simulink model "TestModel_V5_Timing_2024a"  (R2024a)
settings: Solver=FixedStepAuto  StartTime=0.0  StopTime=40  FixedStep=1e-6  RelTol=1e-3
values from neighbouring files (symbols this model uses):
  par_Ctrl_FluxOffset = 0    [Param.m]
  par_Ctrl_MI = 0.99    [Param.m]
  par_Ctrl_SpdRt = 10    [Param.m]
  par_Ctrl_ThetaOffset = 0    [Param.m]
  par_IM_Frated = 50    [Param.m]
  par_IM_IratedPh = 7.9/sqrt(3)    [Param.m]
  par_IM_Lm = 0.527    [Param.m]
  par_IM_Lr = par_IM_Lm + par_IM_Llr    (= 0.5639)    [Param.m]
  par_IM_pp = 2    [Param.m]
  par_IM_Rs = 3.14    [Param.m]
  par_IM_VrmsLL = 400    [Param.m]
  par_uc_Ts = 100e-6    (= 0.0001)    [Param.m]
  pmsm = mcb.getPMSMParameters('Teknic2310P')    [mcb_pmsm_foc_sensorless_f28379d_datascript.m]
  Ts = T_pwm    (= 5e-05)    [mcb_pmsm_foc_sensorless_f28379d_datascript.m]
  Ts_motor = T_pwm/2    (= 2.5e-05)    [mcb_pmsm_foc_sensorless_f28379d_datascript.m]
undefined symbols (not defined in the file or in its folder): DiscIntNeverNeededParam, IM, par_pmsm_FluxLinkage, par_pmsm_Frated, par_pmsm_pp, par_pmsm_Vboost, par_pmsm_VrmsLL
libraries: spsOnDelayLib x24, mcbcontrolslib x11, spsTriangleGeneratorLib x4, autolibim x3, spsCurrentMeasurementLib x2, spsDCVoltageSourceLib x2, spsVoltageMeasurementLib x2, spsTwoLevelConverterLib x2, spsThreePhaseVIMeasurementLib x2, spsSeriesRLCBranchLib x1, sdolib x1, spsUniversalBridgeLib x1
(part 2 of 3)

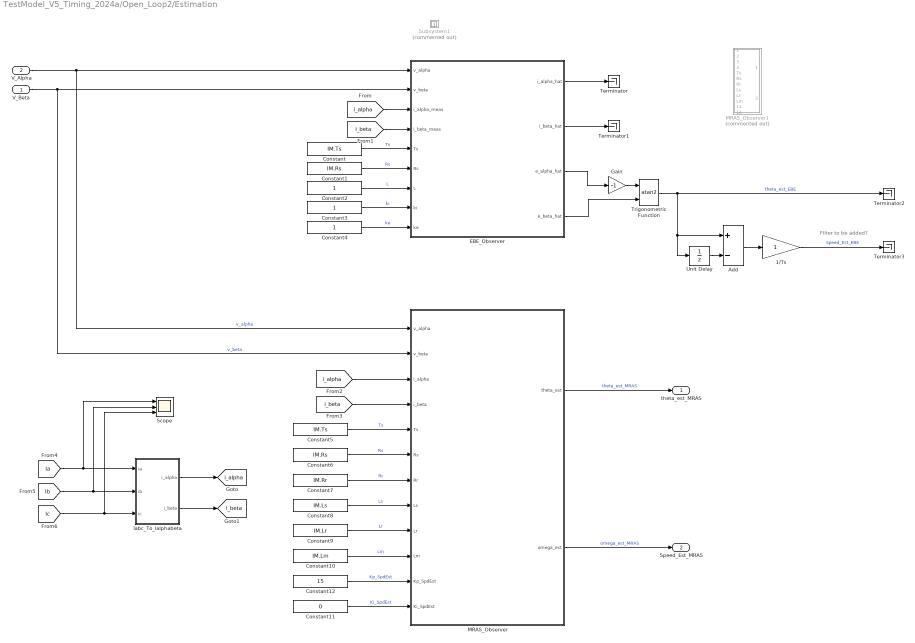
== system TestModel_V5_Timing_2024a/Open_Loop2/Estimation ==
  note: Filter to be added?
  V_Beta : Inport
  V_Alpha : Inport  Port=2
  1/Ts : Gain
  Add : Sum  Inputs=+-
  Constant : Constant  Value=IM.Ts
  Constant1 : Constant  Value=IM.Rs
  Constant10 : Constant  Value=IM.Lm
  Constant11 : Constant  Value=0
  Constant12 : Constant  Value=15
  Constant2 : Constant
  Constant3 : Constant
  Constant4 : Constant
  Constant5 : Constant  Value=IM.Ts
  Constant6 : Constant  Value=IM.Rs
  Constant7 : Constant  Value=IM.Rr
  Constant8 : Constant  Value=IM.Ls
  Constant9 : Constant  Value=IM.Lr
  EBE_Observer : MATLAB Function  TreatAsAtomicUnit=on
  Gain : Gain  Gain=-1
  Iabc_To_Ialphabeta : Subsystem
  MRAS_Observer : MATLAB Function  TreatAsAtomicUnit=on
  MRAS_Observer1 : MATLAB Function  Commented=on  TreatAsAtomicUnit=on
  Scope : Scope  NumInputPorts=3
  Subsystem1 : Subsystem  Commented=on
  Terminator{,1..3} (4 alike) : Terminator
  Trigonometric Function : Trigonometry  Operator=atan2
  Unit Delay : UnitDelay  SampleTime=-1  HasFrameUpgradeWarning=on
  theta_est_MRAS : Outport  VectorParamsAs1DForOutWhenUnconnected=off
  Speed_Est_MRAS : Outport  Port=2  VectorParamsAs1DForOutWhenUnconnected=off
  tag scope: i_alpha=global, i_beta=global
  wires:
  [Ia] -> Scope/1, Iabc_To_Ialphabeta/1(ia)
  [Ib] -> Scope/2, Iabc_To_Ialphabeta/2(ib)
  [Ic] -> Scope/3, Iabc_To_Ialphabeta/3(ic)
  Iabc_To_Ialphabeta/1(i_alpha) -> [i_alpha]
  Iabc_To_Ialphabeta/2(i_beta) -> [i_beta]
  V_Alpha/1 -> MRAS_Observer/1(v_alpha), EBE_Observer/1(v_alpha)  "v_alpha"
  V_Beta/1 -> MRAS_Observer/2(v_beta), EBE_Observer/2(v_beta)  "v_beta"
  Constant/1 -> EBE_Observer/5(Ts)  "Ts"
  Constant1/1 -> EBE_Observer/6(Rs)  "Rs"
  Constant2/1 -> EBE_Observer/7(L)  "L"
  Constant3/1 -> EBE_Observer/8(ki)  "ki"
  Constant4/1 -> EBE_Observer/9(ke)  "ke"
  EBE_Observer/3(e_alpha_hat) -> Gain/1
  Gain/1 -> Trigonometric Function/1
  EBE_Observer/4(e_beta_hat) -> Trigonometric Function/2
  Trigonometric Function/1 -> Terminator2/1, Unit Delay/1, Add/1  "theta_est_EBE"
  Unit Delay/1 -> Add/2
  Add/1 -> 1/Ts/1
  1/Ts/1 -> Terminator3/1  "Speed_Est_EBE"
  EBE_Observer/1(i_alpha_hat) -> Terminator/1
  EBE_Observer/2(i_beta_hat) -> Terminator1/1
  [i_alpha] -> EBE_Observer/3(i_alpha_meas)
  [i_beta] -> EBE_Observer/4(i_beta_meas)
  [i_alpha] -> MRAS_Observer/3(i_alpha)
  [i_beta] -> MRAS_Observer/4(i_beta)
  Constant9/1 -> MRAS_Observer/9(Lr)  "Lr"
  Constant7/1 -> MRAS_Observer/7(Rr)  "Rr"
  Constant6/1 -> MRAS_Observer/6(Rs)  "Rs"
  Constant5/1 -> MRAS_Observer/5(Ts)  "Ts"
  Constant10/1 -> MRAS_Observer/10(Lm)  "Lm"
  Constant12/1 -> MRAS_Observer/11(Kp_SpdEst)  "Kp_SpdEst"
  Constant11/1 -> MRAS_Observer/12(Ki_SpdEst)  "Ki_SpdEst"
  MRAS_Observer/1(theta_est) -> theta_est_MRAS/1  "theta_est_MRAS"
  MRAS_Observer/2(omega_est) -> Speed_Est_MRAS/1  "omega_est_MRAS"
  Constant8/1 -> MRAS_Observer/8(Ls)  "Ls"

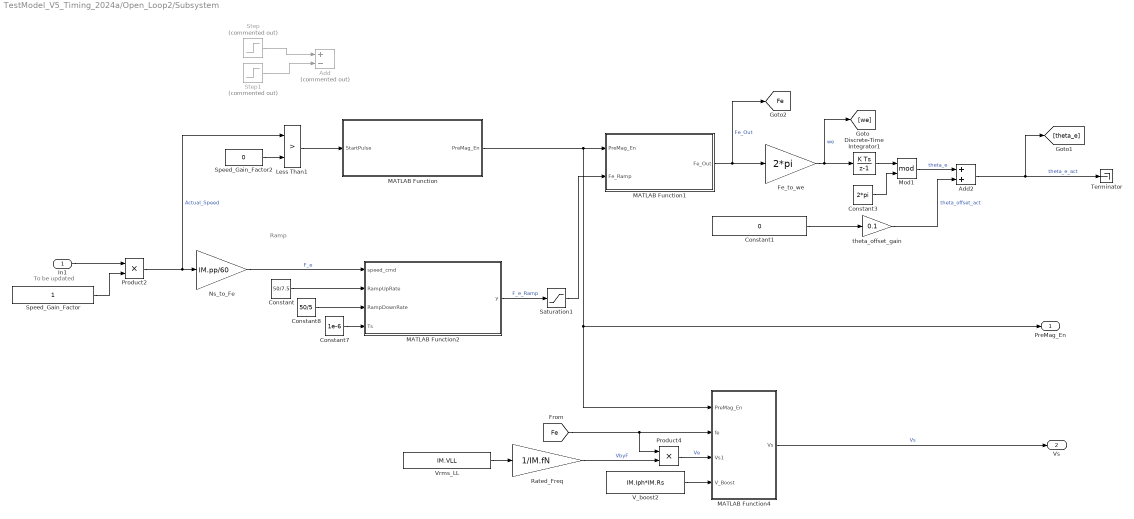
== system TestModel_V5_Timing_2024a/Open_Loop2/Subsystem ==
  note: To be updated
  note: Ramp
  In1 : Inport
  Add : Sum  Commented=on  Inputs=+-
  Add2 : Sum
  Constant : Constant  Value=50/7.5
  Constant1 : Constant  Value=0
  Constant3 : Constant  Value=2*pi  OutDataTypeStr=double
  Constant7 : Constant  Value=1e-6
  Constant8 : Constant  Value=50/5
  Discrete-Time Integrator1 : DiscreteIntegrator  SampleTime=-1  OutDataTypeStr=double  ICPrevOutput=DiscIntNeverNeededParam  ICPrevScaledInput=DiscIntNeverNeededParam
  Fe_to_we : Gain  Gain=2*pi
  Less Than1 : RelationalOperator  Operator=>  OutDataTypeStr=boolean  RndMeth=Simplest  InputSameDT=off
  MATLAB Function : MATLAB Function  TreatAsAtomicUnit=on
  MATLAB Function1 : MATLAB Function  TreatAsAtomicUnit=on
  MATLAB Function2 : MATLAB Function  TreatAsAtomicUnit=on
  MATLAB Function4 : MATLAB Function  TreatAsAtomicUnit=on
  Mod1 : Math  Operator=mod
  Ns_to_Fe : Gain  Gain=IM.pp/60
  Product2 : Product
  Product4 : Product
  Rated_Freq : Gain  Gain=1/IM.fN  ParamDataTypeStr=double  OutDataTypeStr=double
  Saturation1 : Saturate  UpperLimit=50  LowerLimit=0
  Speed_Gain_Factor : Constant
  Speed_Gain_Factor2 : Constant  Value=0
  Step : Step  Commented=on
  Step1 : Step  Commented=on  Time=1.2
  Terminator : Terminator
  V_boost2 : Constant  Value=IM.Iph*IM.Rs
  Vrms_LL : Constant  Value=IM.VLL  OutDataTypeStr=double
  theta_offset_gain : Gain  Gain=0.1
  PreMag_En : Outport  VectorParamsAs1DForOutWhenUnconnected=off
  Vs : Outport  Port=2  VectorParamsAs1DForOutWhenUnconnected=off
  tag scope: Fe=global
  wires:
  Step1/1 -> Add/2
  Add2/1 -> Terminator/1, [theta_e]  "theta_e_act"
  Discrete-Time Integrator1/1 -> Mod1/1
  Product2/1 -> Ns_to_Fe/1, Less Than1/1  "Actual_Speed"
  MATLAB Function/1(PreMag_En) -> MATLAB Function4/1(PreMag_En), PreMag_En/1, MATLAB Function1/1(PreMag_En)
  [Fe] -> MATLAB Function4/2(fe), Product4/1
  Product4/1 -> MATLAB Function4/3(Vs1)  "Ve"
  Constant1/1 -> theta_offset_gain/1
  Rated_Freq/1 -> Product4/2  "VbyF"
  V_boost2/1 -> MATLAB Function4/4(V_Boost)
  MATLAB Function1/1(Fe_Out) -> [Fe], Fe_to_we/1  "Fe_Out"
  Constant/1 -> MATLAB Function2/2(RampUpRate)
  Fe_to_we/1 -> Discrete-Time Integrator1/1, [we]  "we"
  Constant7/1 -> MATLAB Function2/4(Ts)
  Less Than1/1 -> MATLAB Function/1(StartPulse)
  Saturation1/1 -> MATLAB Function1/2(Fe_Ramp)
  Ns_to_Fe/1 -> MATLAB Function2/1(speed_cmd)  "F_e"
  Step/1 -> Add/1
  Speed_Gain_Factor2/1 -> Less Than1/2
  Speed_Gain_Factor/1 -> Product2/2
  Constant8/1 -> MATLAB Function2/3(RampDownRate)
  MATLAB Function4/1(Vs) -> Vs/1  "Vs"
  Mod1/1 -> Add2/1  "theta_e"
  MATLAB Function2/1(y) -> Saturation1/1  "F_e_Ramp"
  Constant3/1 -> Mod1/2
  theta_offset_gain/1 -> Add2/2  "theta_offset_act"
  Vrms_LL/1 -> Rated_Freq/1
  In1/1 -> Product2/1

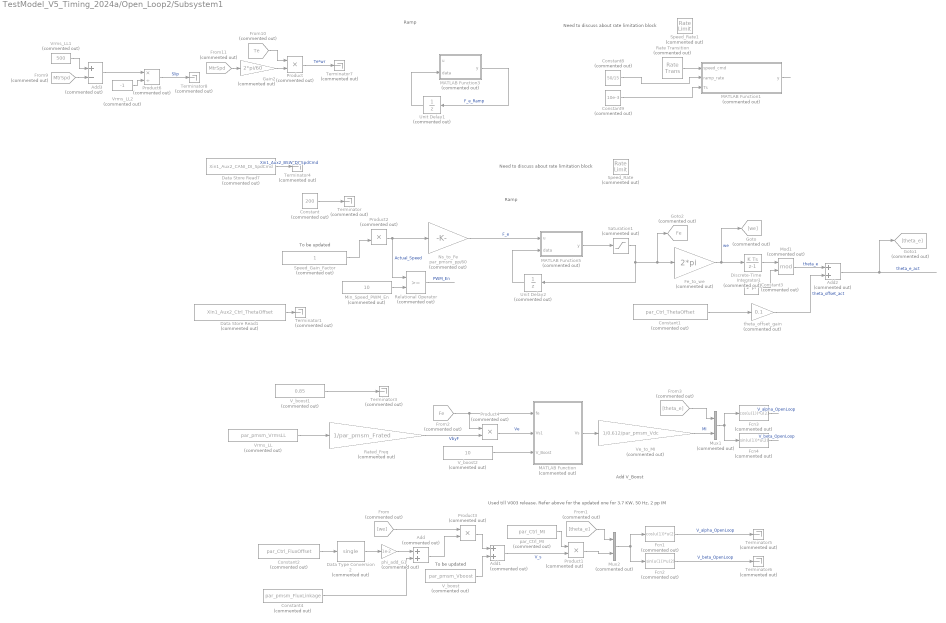
== system TestModel_V5_Timing_2024a/Open_Loop2/Subsystem1 ==
  note: Add V_Boost
  note: Used till V003 release. Refer above for the updated one for 3.7 KW, 50 Hz, 2 pp IM
  note: Ramp
  note: Need to discuss about rate limitation block
  note: To be updated
  note: To be updated
  note: Need to discuss about rate limitation block
  note: Ramp
  Add : Sum  Commented=on
  Add1 : Sum  Commented=on
  Add2 : Sum  Commented=on
  Add3 : Sum  Commented=on  Inputs=+-
  Constant : Constant  Commented=on  Value=200
  Constant1 : Constant  Commented=on  Value=par_Ctrl_ThetaOffset
  Constant2 : Constant  Commented=on  Value=par_Ctrl_FluxOffset
  Constant3 : Constant  Commented=on  Value=2*pi  OutDataTypeStr=double
  Constant4 : Constant  Commented=on  Value=par_pmsm_FluxLinkage  OutDataTypeStr=double
  Constant8 : Constant  Commented=on  Value=50/15
  Constant9 : Constant  Commented=on  Value=10e-3
  Data Store Read1 : DataStoreRead  Commented=on  DataStoreName=Xin1_Aux2_Ctrl_ThetaOffset  IndexOptions=Index vector (dialog)  Indices=1  OutputSizes=1
  Data Store Read7 : DataStoreRead  Commented=on  DataStoreName=Xin1_Aux2_CANI_DI_SpdCmd  IndexOptions=Index vector (dialog)  Indices=1  OutputSizes=1
  Data Type Conversion2 : DataTypeConversion  Commented=on  OutDataTypeStr=single  SaturateOnIntegerOverflow=off  RndMeth=Floor
  Discrete-Time Integrator1 : DiscreteIntegrator  Commented=on  SampleTime=-1  OutDataTypeStr=double  ICPrevOutput=DiscIntNeverNeededParam  ICPrevScaledInput=DiscIntNeverNeededParam
  Fcn1 : Fcn  Commented=on  Expr=cos(u(1))*u(2)
  Fcn2 : Fcn  Commented=on  Expr=sin(u(1))*u(2)
  Fcn3 : Fcn  Commented=on  Expr=cos(u(1))*u(2)
  Fcn4 : Fcn  Commented=on  Expr=sin(u(1))*u(2)
  Fe_to_we : Gain  Commented=on  Gain=2*pi
  From : From  Commented=on  GotoTag=we
  From1 : From  Commented=on  GotoTag=theta_e
  From10 : From  Commented=on  GotoTag=Te
  From11 : From  Commented=on  GotoTag=MtrSpd
  From2 : From  Commented=on  GotoTag=Fe  TagVisibility=global
  From3 : From  Commented=on  GotoTag=theta_e
  From9 : From  Commented=on  GotoTag=MtrSpd
  Gain2 : Gain  Commented=on  Gain=2*pi/60
  Goto : Goto  Commented=on  GotoTag=we
  Goto1 : Goto  Commented=on  GotoTag=theta_e
  Goto2 : Goto  Commented=on  GotoTag=Fe  TagVisibility=global
  MATLAB Function : MATLAB Function  Commented=on  TreatAsAtomicUnit=on
  MATLAB Function1 : MATLAB Function  Commented=on  TreatAsAtomicUnit=on
  MATLAB Function3 : MATLAB Function  Commented=on  TreatAsAtomicUnit=on
  MATLAB Function5 : MATLAB Function  Commented=on  TreatAsAtomicUnit=on
  Min_Speed_PWM_En : Constant  Commented=on  Value=10
  Mod1 : Math  Commented=on  Operator=mod
  Mux1 : Mux  Commented=on  Inputs=2
  Mux2 : Mux  Commented=on  Inputs=2
  Ns_to_Fe : Gain  Commented=on  Gain=par_pmsm_pp/60
  Product{,1..4} (5 alike) : Product  Commented=on
  Product6 : Product  Commented=on  Inputs=*/
  Rate Transition : RateTransition  Commented=on  OutPortSampleTime=10e-3
  Rated_Freq : Gain  Commented=on  Gain=1/par_pmsm_Frated  ParamDataTypeStr=double  OutDataTypeStr=double
  Relational Operator : RelationalOperator  Commented=on  OutDataTypeStr=boolean  RndMeth=Simplest  InputSameDT=off
  Saturation1 : Saturate  Commented=on  UpperLimit=50  LowerLimit=0
  Speed_Gain_Factor : Constant  Commented=on
  Speed_Rate : RateLimiter  Commented=on  RisingSlewLimit=par_Ctrl_SpdRt  FallingSlewLimit=-par_Ctrl_SpdRt  SampleTimeMode=inherited
  Speed_Rate1 : RateLimiter  Commented=on  RisingSlewLimit=par_Ctrl_SpdRt  FallingSlewLimit=-par_Ctrl_SpdRt  SampleTimeMode=inherited
  Terminator{,1,3..8} (8 alike) : Terminator  Commented=on
  Unit Delay1 : UnitDelay  Commented=on  SampleTime=-1  HasFrameUpgradeWarning=on
  Unit Delay2 : UnitDelay  Commented=on  SampleTime=-1  HasFrameUpgradeWarning=on
  V_boost : Constant  Commented=on  Value=par_pmsm_Vboost
  V_boost1 : Constant  Commented=on  Value=0.85
  V_boost2 : Constant  Commented=on  Value=10
  Ve_to_MI : Gain  Commented=on  Gain=1/0.612/par_pmsm_Vdc  ParamDataTypeStr=double  OutDataTypeStr=double
  Vrms_LL : Constant  Commented=on  Value=par_pmsm_VrmsLL  OutDataTypeStr=double
  Vrms_LL1 : Constant  Commented=on  Value=500  OutDataTypeStr=double  SampleTime=-1
  Vrms_LL2 : Constant  Commented=on  Value=-1  OutDataTypeStr=double
  par_Ctrl_MI : Constant  Commented=on  Value=par_Ctrl_MI
  phi_add_G1 : Gain  Commented=on  Gain=1e-2  ParamDataTypeStr=double  OutDataTypeStr=double
  theta_offset_gain : Gain  Commented=on  Gain=0.1
  wires:
  phi_add_G1/1 -> Add/1
  Add2/1 -> Goto1/1  "theta_e_act"
  Relational Operator/1 -> ?  "PWM_En"
  Fcn1/1 -> Terminator5/1  "V_alpha_OpenLoop"
  Add/1 -> Product3/2
  Product1/1 -> Mux2/2
  Saturation1/1 -> Unit Delay2/1, Goto2/1, Fe_to_we/1
  Constant3/1 -> Mod1/2
  Product2/1 -> Relational Operator/1, Ns_to_Fe/1  "Actual_Speed"
  Constant4/1 -> Add/2
  Fcn2/1 -> Terminator6/1  "V_beta_OpenLoop"
  MATLAB Function3/1(y) -> Unit Delay1/1  "F_e_Ramp"
  Vrms_LL/1 -> Rated_Freq/1
  Constant/1 -> Terminator/1
  Constant9/1 -> MATLAB Function1/3(Ts)
  Mux1/1 -> Fcn4/1, Fcn3/1
  V_boost/1 -> Add1/2
  theta_offset_gain/1 -> Add2/2  "theta_offset_act"
  par_Ctrl_MI/1 -> Product1/1
  Data Store Read1/1 -> Terminator1/1
  Fe_to_we/1 -> Discrete-Time Integrator1/1, Goto/1  "we"
  Ns_to_Fe/1 -> MATLAB Function5/1(u)  "F_e"
  Add1/1 -> Product1/2  "V_s"
  Product3/1 -> Add1/1
  ? -> Product2/1  "Xin1_Aux1_CANI_DI_SpdCmd"
  ? -> Rate Transition/1
  Constant8/1 -> MATLAB Function1/2(ramp_rate)
  Speed_Gain_Factor/1 -> Product2/2
  Fcn4/1 -> ?  "V_beta_OpenLoop"
  V_boost1/1 -> Terminator3/1
  Mod1/1 -> Add2/1  "theta_e"
  Data Store Read7/1 -> Terminator4/1  "Xin1_Aux2_BSW_DI_SpdCmd"
  From1/1 -> Mux2/1
  Fcn3/1 -> ?  "V_alpha_OpenLoop"
  Product4/1 -> MATLAB Function/2(Vs1)  "Ve"
  Mux2/1 -> Fcn2/1, Fcn1/1
  From2/1 -> Product4/1, MATLAB Function/1(fe)
  Discrete-Time Integrator1/1 -> Mod1/1
  Unit Delay1/1 -> MATLAB Function3/2(data)
  Constant2/1 -> Data Type Conversion2/1
  Ve_to_MI/1 -> Mux1/2  "MI"
  Data Type Conversion2/1 -> phi_add_G1/1
  MATLAB Function5/1(y) -> Saturation1/1
  Min_Speed_PWM_En/1 -> Relational Operator/2
  From3/1 -> Mux1/1
  Rate Transition/1 -> MATLAB Function1/1(speed_cmd)
  Rated_Freq/1 -> Product4/2  "VbyF"
  MATLAB Function1/1(y) -> ?
  Constant1/1 -> theta_offset_gain/1
  Unit Delay2/1 -> MATLAB Function5/2(data)
  MATLAB Function/1(Vs) -> Ve_to_MI/1
  V_boost2/1 -> MATLAB Function/3(V_Boost)
  From/1 -> Product3/1
  ? -> MATLAB Function3/1(u)
  Vrms_LL1/1 -> Add3/1
  From9/1 -> Add3/2
  From11/1 -> Gain2/1
  Product6/1 -> Terminator8/1  "Slip"
  From10/1 -> Product/1
  Add3/1 -> Product6/1
  Gain2/1 -> Product/2
  Vrms_LL2/1 -> Product6/2
  Product/1 -> Terminator7/1  "Te*wr"

== system TestModel_V5_Timing_2024a/Subsystem/Brake ==
  Constant : Constant  Commented=on  Value=pmsm.LdTrq
  Data Type Conversion : DataTypeConversion  Commented=on  OutDataTypeStr=single  SaturateOnIntegerOverflow=off  RndMeth=Floor
  IIR Filter : mcbcontrolslib/IIR Filter  VariantControl=Low Pass Filter  VariantSelect=Low-pass  FilterConstantInputType=Specify via dialog  Filter_constant=0.001  InitialOutput=Specify via dialog  InitialOutputValue=0  ExternalReset=none  advancedSettings=off  Ts=50e-6  cutOff_freq=3.1863
  T_load : Step  Time=2.5  Before=pmsm.T_rated*0  After=pmsm.T_rated*0.1  SampleTime=Ts_motor
  T_load1 : Step  Commented=on  Time=2.5  Before=pmsm.T_rated*0.1  After=pmsm.T_rated*0.5  SampleTime=Ts_motor
  Terminator : Terminator
  Out1 : Outport
  wires:
  Constant/1 -> Terminator/1
  T_load/1 -> IIR Filter/1
  IIR Filter/1 -> Out1/1

== system TestModel_V5_Timing_2024a/Subsystem1/Subsystem ==
  fe : Inport
  fb_teta : Inport  Port=2
  2pi : Constant  Value=2*pi
  Discrete-Time Integrator : DiscreteIntegrator  ExternalReset=rising  SampleTime=-1  LimitOutput=on  UpperSaturationLimit=2*pi  LowerSaturationLimit=0  ICPrevOutput=DiscIntNeverNeededParam  ICPrevScaledInput=DiscIntNeverNeededParam
  Equal : RelationalOperator  OutDataTypeStr=boolean  RndMeth=Simplest  InputSameDT=off
  tetaOL : Outport
  wires:
  fb_teta/1 -> Equal/1
  Equal/1 -> Discrete-Time Integrator/2
  2pi/1 -> Equal/2
  Discrete-Time Integrator/1 -> tetaOL/1  "tetaOL"
  fe/1 -> Discrete-Time Integrator/1

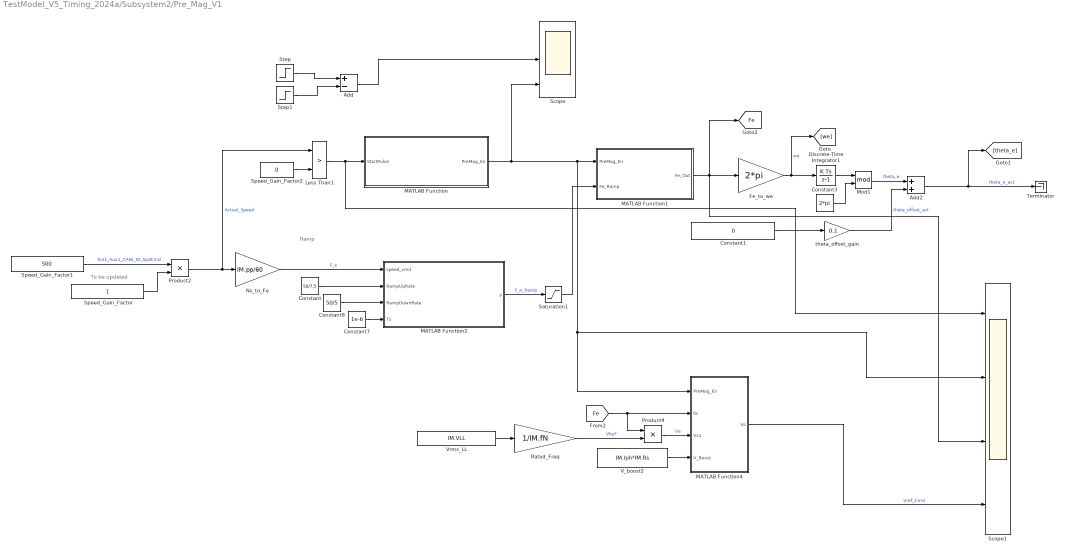
== system TestModel_V5_Timing_2024a/Subsystem2/Pre_Mag_V1 ==
  note: To be updated
  note: Ramp
  Add : Sum  Inputs=+-
  Add2 : Sum
  Constant : Constant  Value=50/7.5
  Constant1 : Constant  Value=0
  Constant3 : Constant  Value=2*pi  OutDataTypeStr=double
  Constant7 : Constant  Value=1e-6
  Constant8 : Constant  Value=50/5
  Discrete-Time Integrator1 : DiscreteIntegrator  SampleTime=-1  OutDataTypeStr=double  ICPrevOutput=DiscIntNeverNeededParam  ICPrevScaledInput=DiscIntNeverNeededParam
  Fe_to_we : Gain  Gain=2*pi
  Less Than1 : RelationalOperator  Operator=>  OutDataTypeStr=boolean  RndMeth=Simplest  InputSameDT=off
  MATLAB Function : MATLAB Function  TreatAsAtomicUnit=on
  MATLAB Function1 : MATLAB Function  TreatAsAtomicUnit=on
  MATLAB Function2 : MATLAB Function  TreatAsAtomicUnit=on
  MATLAB Function4 : MATLAB Function  TreatAsAtomicUnit=on
  Mod1 : Math  Operator=mod
  Ns_to_Fe : Gain  Gain=IM.pp/60
  Product2 : Product
  Product4 : Product
  Rated_Freq : Gain  Gain=1/IM.fN  ParamDataTypeStr=double  OutDataTypeStr=double
  Saturation1 : Saturate  UpperLimit=50  LowerLimit=0
  Scope : Scope  NumInputPorts=3
  Scope1 : Scope  NumInputPorts=4
  Speed_Gain_Factor : Constant
  Speed_Gain_Factor1 : Constant  Value=500
  Speed_Gain_Factor2 : Constant  Value=0
  Step : Step
  Step1 : Step  Time=1.2
  Terminator : Terminator
  V_boost2 : Constant  Value=IM.Iph*IM.Rs
  Vrms_LL : Constant  Value=IM.VLL  OutDataTypeStr=double
  theta_offset_gain : Gain  Gain=0.1
  tag scope: Fe=global
  wires:
  Step1/1 -> Add/2
  Add2/1 -> Terminator/1, [theta_e]  "theta_e_act"
  Discrete-Time Integrator1/1 -> Mod1/1
  Product2/1 -> Ns_to_Fe/1, Less Than1/1  "Actual_Speed"
  MATLAB Function/1(PreMag_En) -> Scope/3, Scope1/2, MATLAB Function4/1(PreMag_En), MATLAB Function1/1(PreMag_En)
  [Fe] -> MATLAB Function4/2(fe), Product4/1
  Product4/1 -> MATLAB Function4/3(Vs1)  "Ve"
  Constant1/1 -> theta_offset_gain/1
  Rated_Freq/1 -> Product4/2  "VbyF"
  V_boost2/1 -> MATLAB Function4/4(V_Boost)
  MATLAB Function1/1(Fe_Out) -> Scope1/3, [Fe], Fe_to_we/1
  Constant/1 -> MATLAB Function2/2(RampUpRate)
  Fe_to_we/1 -> Discrete-Time Integrator1/1, [we]  "we"
  Constant7/1 -> MATLAB Function2/4(Ts)
  Less Than1/1 -> MATLAB Function/1(StartPulse), Scope1/1
  Saturation1/1 -> MATLAB Function1/2(Fe_Ramp)
  Ns_to_Fe/1 -> MATLAB Function2/1(speed_cmd)  "F_e"
  Step/1 -> Add/1
  Add/1 -> Scope/2
  Speed_Gain_Factor2/1 -> Less Than1/2
  Speed_Gain_Factor1/1 -> Product2/1  "Xin1_Aux1_CANI_DI_SpdCmd"
  Speed_Gain_Factor/1 -> Product2/2
  Constant8/1 -> MATLAB Function2/3(RampDownRate)
  MATLAB Function4/1(Vs) -> Scope1/4  "Vref_Cmd"
  Mod1/1 -> Add2/1  "theta_e"
  MATLAB Function2/1(y) -> Saturation1/1  "F_e_Ramp"
  Constant3/1 -> Mod1/2
  theta_offset_gain/1 -> Add2/2  "theta_offset_act"
  Vrms_LL/1 -> Rated_Freq/1

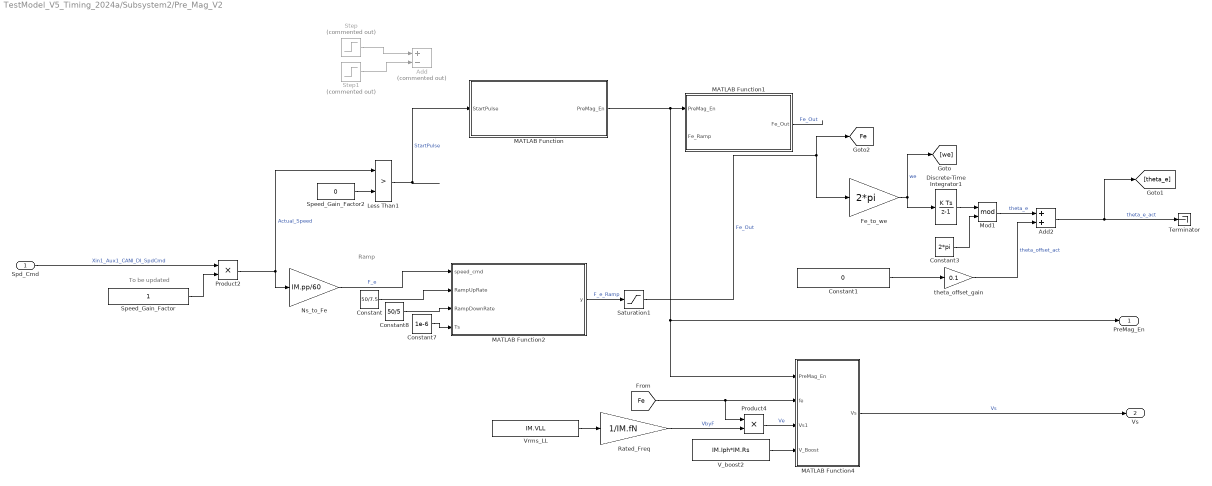
== system TestModel_V5_Timing_2024a/Subsystem2/Pre_Mag_V2 ==
  note: To be updated
  note: Ramp
  Spd_Cmd : Inport
  Add : Sum  Commented=on  Inputs=+-
  Add2 : Sum
  Constant : Constant  Value=50/7.5
  Constant1 : Constant  Value=0
  Constant3 : Constant  Value=2*pi  OutDataTypeStr=double
  Constant7 : Constant  Value=1e-6
  Constant8 : Constant  Value=50/5
  Discrete-Time Integrator1 : DiscreteIntegrator  SampleTime=-1  OutDataTypeStr=double  ICPrevOutput=DiscIntNeverNeededParam  ICPrevScaledInput=DiscIntNeverNeededParam
  Fe_to_we : Gain  Gain=2*pi
  Less Than1 : RelationalOperator  Operator=>  OutDataTypeStr=boolean  RndMeth=Simplest  InputSameDT=off
  MATLAB Function : MATLAB Function  TreatAsAtomicUnit=on
  MATLAB Function1 : MATLAB Function  TreatAsAtomicUnit=on
  MATLAB Function2 : MATLAB Function  TreatAsAtomicUnit=on
  MATLAB Function4 : MATLAB Function  TreatAsAtomicUnit=on
  Mod1 : Math  Operator=mod
  Ns_to_Fe : Gain  Gain=IM.pp/60
  Product2 : Product
  Product4 : Product
  Rated_Freq : Gain  Gain=1/IM.fN  ParamDataTypeStr=double  OutDataTypeStr=double
  Saturation1 : Saturate  UpperLimit=50  LowerLimit=0
  Speed_Gain_Factor : Constant
  Speed_Gain_Factor2 : Constant  Value=0
  Step : Step  Commented=on
  Step1 : Step  Commented=on  Time=1.2
  Terminator : Terminator
  V_boost2 : Constant  Value=IM.Iph*IM.Rs
  Vrms_LL : Constant  Value=IM.VLL  OutDataTypeStr=double
  theta_offset_gain : Gain  Gain=0.1
  PreMag_En : Outport  VectorParamsAs1DForOutWhenUnconnected=off
  Vs : Outport  Port=2  VectorParamsAs1DForOutWhenUnconnected=off
  tag scope: Fe=global
  wires:
  Step1/1 -> Add/2
  Add2/1 -> [theta_e], Terminator/1  "theta_e_act"
  Discrete-Time Integrator1/1 -> Mod1/1
  Product2/1 -> Ns_to_Fe/1, Less Than1/1  "Actual_Speed"
  MATLAB Function/1(PreMag_En) -> MATLAB Function4/1(PreMag_En), PreMag_En/1, MATLAB Function1/1(PreMag_En)
  [Fe] -> MATLAB Function4/2(fe), Product4/1
  Product4/1 -> MATLAB Function4/3(Vs1)  "Ve"
  Constant1/1 -> theta_offset_gain/1
  Rated_Freq/1 -> Product4/2  "VbyF"
  V_boost2/1 -> MATLAB Function4/4(V_Boost)
  Saturation1/1 -> [Fe], Fe_to_we/1  "Fe_Out"
  Constant/1 -> MATLAB Function2/2(RampUpRate)
  Fe_to_we/1 -> [we], Discrete-Time Integrator1/1  "we"
  Constant7/1 -> MATLAB Function2/4(Ts)
  Less Than1/1 -> MATLAB Function/1(StartPulse)  "StartPulse"
  Ns_to_Fe/1 -> MATLAB Function2/1(speed_cmd)  "F_e"
  Step/1 -> Add/1
  Speed_Gain_Factor2/1 -> Less Than1/2
  Speed_Gain_Factor/1 -> Product2/2
  Constant8/1 -> MATLAB Function2/3(RampDownRate)
  MATLAB Function4/1(Vs) -> Vs/1  "Vs"
  Mod1/1 -> Add2/1  "theta_e"
  MATLAB Function2/1(y) -> Saturation1/1  "F_e_Ramp"
  Constant3/1 -> Mod1/2
  theta_offset_gain/1 -> Add2/2  "theta_offset_act"
  Vrms_LL/1 -> Rated_Freq/1
  Spd_Cmd/1 -> Product2/1  "Xin1_Aux1_CANI_DI_SpdCmd"
  MATLAB Function1/1(Fe_Out) -> ?  "Fe_Out"

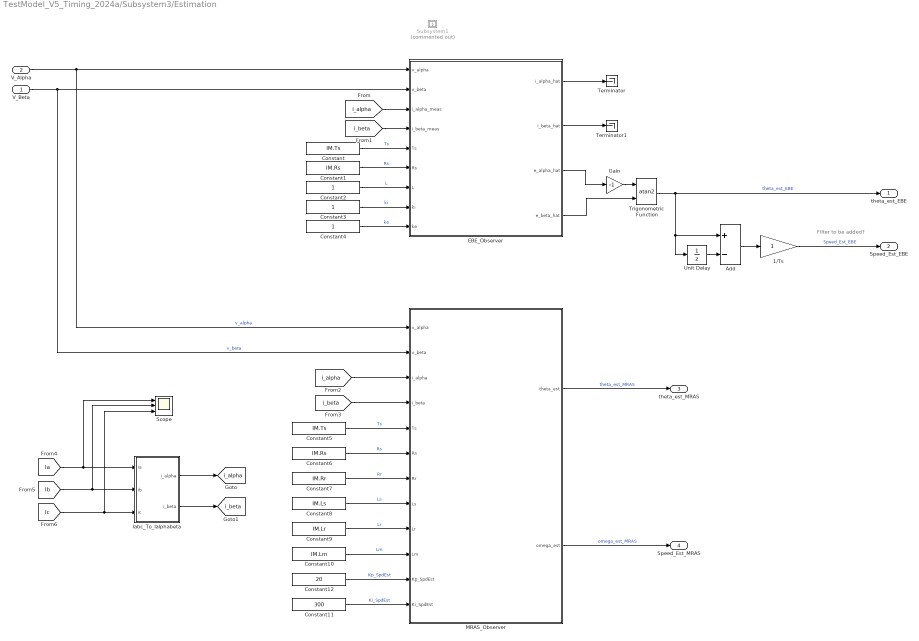
== system TestModel_V5_Timing_2024a/Subsystem3/Estimation ==
  note: Filter to be added?
  V_Beta : Inport
  V_Alpha : Inport  Port=2
  1/Ts : Gain
  Add : Sum  Inputs=+-
  Constant : Constant  Value=IM.Ts
  Constant1 : Constant  Value=IM.Rs
  Constant10 : Constant  Value=IM.Lm
  Constant11 : Constant  Value=300
  Constant12 : Constant  Value=20
  Constant2 : Constant
  Constant3 : Constant
  Constant4 : Constant
  Constant5 : Constant  Value=IM.Ts
  Constant6 : Constant  Value=IM.Rs
  Constant7 : Constant  Value=IM.Rr
  Constant8 : Constant  Value=IM.Ls
  Constant9 : Constant  Value=IM.Lr
  EBE_Observer : MATLAB Function  TreatAsAtomicUnit=on
  Gain : Gain  Gain=-1
  Iabc_To_Ialphabeta : Subsystem
  MRAS_Observer : MATLAB Function  TreatAsAtomicUnit=on
  Scope : Scope  NumInputPorts=3
  Subsystem1 : Subsystem  Commented=on
  Terminator : Terminator
  Terminator1 : Terminator
  Trigonometric Function : Trigonometry  Operator=atan2
  Unit Delay : UnitDelay  SampleTime=-1  HasFrameUpgradeWarning=on
  theta_est_EBE : Outport  VectorParamsAs1DForOutWhenUnconnected=off
  Speed_Est_EBE : Outport  Port=2  VectorParamsAs1DForOutWhenUnconnected=off
  theta_est_MRAS : Outport  Port=3  VectorParamsAs1DForOutWhenUnconnected=off
  Speed_Est_MRAS : Outport  Port=4  VectorParamsAs1DForOutWhenUnconnected=off
  tag scope: i_alpha=global, i_beta=global
  wires:
  [Ia] -> Scope/1, Iabc_To_Ialphabeta/1(ia)
  [Ib] -> Scope/2, Iabc_To_Ialphabeta/2(ib)
  [Ic] -> Scope/3, Iabc_To_Ialphabeta/3(ic)
  Iabc_To_Ialphabeta/1(i_alpha) -> [i_alpha]
  Iabc_To_Ialphabeta/2(i_beta) -> [i_beta]
  V_Alpha/1 -> MRAS_Observer/1(v_alpha), EBE_Observer/1(v_alpha)  "v_alpha"
  V_Beta/1 -> MRAS_Observer/2(v_beta), EBE_Observer/2(v_beta)  "v_beta"
  Constant/1 -> EBE_Observer/5(Ts)  "Ts"
  Constant1/1 -> EBE_Observer/6(Rs)  "Rs"
  Constant2/1 -> EBE_Observer/7(L)  "L"
  Constant3/1 -> EBE_Observer/8(ki)  "ki"
  Constant4/1 -> EBE_Observer/9(ke)  "ke"
  EBE_Observer/3(e_alpha_hat) -> Gain/1
  Gain/1 -> Trigonometric Function/1
  EBE_Observer/4(e_beta_hat) -> Trigonometric Function/2
  Trigonometric Function/1 -> Unit Delay/1, Add/1, theta_est_EBE/1  "theta_est_EBE"
  Unit Delay/1 -> Add/2
  Add/1 -> 1/Ts/1
  1/Ts/1 -> Speed_Est_EBE/1  "Speed_Est_EBE"
  EBE_Observer/1(i_alpha_hat) -> Terminator/1
  EBE_Observer/2(i_beta_hat) -> Terminator1/1
  [i_alpha] -> EBE_Observer/3(i_alpha_meas)
  [i_beta] -> EBE_Observer/4(i_beta_meas)
  [i_alpha] -> MRAS_Observer/3(i_alpha)
  [i_beta] -> MRAS_Observer/4(i_beta)
  Constant9/1 -> MRAS_Observer/9(Lr)  "Lr"
  Constant7/1 -> MRAS_Observer/7(Rr)  "Rr"
  Constant6/1 -> MRAS_Observer/6(Rs)  "Rs"
  Constant5/1 -> MRAS_Observer/5(Ts)  "Ts"
  Constant10/1 -> MRAS_Observer/10(Lm)  "Lm"
  Constant12/1 -> MRAS_Observer/11(Kp_SpdEst)  "Kp_SpdEst"
  Constant11/1 -> MRAS_Observer/12(Ki_SpdEst)  "Ki_SpdEst"
  MRAS_Observer/1(theta_est) -> theta_est_MRAS/1  "theta_est_MRAS"
  MRAS_Observer/2(omega_est) -> Speed_Est_MRAS/1  "omega_est_MRAS"
  Constant8/1 -> MRAS_Observer/8(Ls)  "Ls"

== system TestModel_V5_Timing_2024a/Open_Loop2/Estimation/Iabc_To_Ialphabeta ==
  ia : Inport
  ib : Inport  Port=2
  ic : Inport  Port=3
  Add : Sum  Inputs=+--
  Add1 : Sum  Inputs=-+
  Clarke Transform : mcbcontrolslib/Clarke Transform  VariantControl=Variant2  EnPowerInv=off  PhaseInput=Two inputs
      settings: LibrarySourceBlock=mcbhdllib/Controls/Math Transforms/Clarke Transform
  Gain : Gain  Gain=0.5
  Gain1 : Gain  Gain=0.5
  Gain2 : Gain  Gain=2/3
  Gain3 : Gain  Gain=sqrt(3)/2
  Gain4 : Gain  Gain=sqrt(3)/2
  Gain5 : Gain  Gain=2/3
  i_alpha : Outport
  i_beta : Outport  Port=2
  wires:
  Gain3/1 -> Add1/1
  Gain/1 -> Add/2
  ib/1 -> Gain4/1, Gain/1
  Gain5/1 -> i_beta/1  "i_beta"
  ic/1 -> Gain3/1, Gain1/1
  Gain1/1 -> Add/3
  Add1/1 -> Gain5/1
  Add/1 -> Gain2/1
  Gain4/1 -> Add1/2  "i_alpha"
  ia/1 -> Add/1
  Gain2/1 -> i_alpha/1  "i_alpha"

== system TestModel_V5_Timing_2024a/Open_Loop2/Estimation/Subsystem1 ==
  In Bus Element : Inport  PortName=Ctrl_ScaledISR_In  Element=signal1
  Bus Selector : BusSelector  OutputSignals=signal1,signal2
  Fcn : Fcn  Expr=sin(u(1)*exp(2.3*(-u(2))))
  Iabc_To_Ialphabeta : Subsystem
  Park Transform : mcbcontrolslib/Park Transform  AxisAlignment=D-axis  PhaseInput=Two inputs  ThetaInput=Sine and Cosine electrical position  AngleInput=Per-unit  N_points=1024
      settings: LibrarySourceBlock=mcbhdllib/Controls/Math Transforms/Park Transform
  Pos_Est : Subsystem
  Subsystem : Subsystem
  Terminator : Terminator
  V_AlphaBeta : Subsystem
  di/dt : Subsystem
  emf_AlphaBeta : Subsystem
  Out Bus Element : Outport  PortName=Position_Est  Element=signal1
  Out Bus Element1 : Outport  Port=2  PortName=Speed_Est  Element=signal1
  wires:
  di/dt/1(dia/dt) -> emf_AlphaBeta/3(dia/dt)
  Iabc_To_Ialphabeta/1(i_alpha) -> di/dt/1(i_alpha), [i_alpha]
  emf_AlphaBeta/2(emf_beta) -> Pos_Est/2(emf_beta)
  di/dt/2(dib/dt) -> emf_AlphaBeta/4(dib/dt)
  emf_AlphaBeta/1(emf_alpha) -> Pos_Est/1(emf_alpha)
  V_AlphaBeta/3(V_C) -> Terminator/1
  [i_beta] -> emf_AlphaBeta/2(i_beta)
  [i_alpha] -> emf_AlphaBeta/1(i_alpha)
  V_AlphaBeta/2(V_beta) -> emf_AlphaBeta/6(v_beta)
  ? -> V_AlphaBeta/3(D_b)
  ? -> V_AlphaBeta/1(V_DC)
  V_AlphaBeta/1(V_alpha) -> emf_AlphaBeta/5(v_alpha)
  Iabc_To_Ialphabeta/2(i_beta) -> di/dt/2(i_beta), [i_beta]
  Park Transform/2 -> ?
  Fcn/1 -> ?
  ? -> Iabc_To_Ialphabeta/2(ib)
  Pos_Est/1(Position) -> ?
  ? -> Iabc_To_Ialphabeta/3(ic)
  ? -> Iabc_To_Ialphabeta/1(ia)
  ? -> V_AlphaBeta/4(D_c)
  ? -> V_AlphaBeta/2(D_a)
  Bus Selector/1 -> ?  "<signal1>"
  ? -> Fcn/1
  Park Transform/1 -> ?
  Bus Selector/2 -> ?  "<signal2>"

== system TestModel_V5_Timing_2024a/Subsystem3/Estimation/Iabc_To_Ialphabeta ==
  ia : Inport
  ib : Inport  Port=2
  ic : Inport  Port=3
  Add : Sum  Inputs=+--
  Add1 : Sum  Inputs=-+
  Clarke Transform : mcbcontrolslib/Clarke Transform  VariantControl=Variant2  EnPowerInv=off  PhaseInput=Two inputs
      settings: LibrarySourceBlock=mcbhdllib/Controls/Math Transforms/Clarke Transform
  Gain : Gain  Gain=0.5
  Gain1 : Gain  Gain=0.5
  Gain2 : Gain  Gain=2/3
  Gain3 : Gain  Gain=sqrt(3)/2
  Gain4 : Gain  Gain=sqrt(3)/2
  Gain5 : Gain  Gain=2/3
  i_alpha : Outport
  i_beta : Outport  Port=2
  wires:
  Gain3/1 -> Add1/1
  Gain/1 -> Add/2
  ib/1 -> Gain4/1, Gain/1
  Gain5/1 -> i_beta/1  "i_beta"
  ic/1 -> Gain3/1, Gain1/1
  Gain1/1 -> Add/3
  Add1/1 -> Gain5/1
  Add/1 -> Gain2/1
  Gain4/1 -> Add1/2  "i_alpha"
  ia/1 -> Add/1
  Gain2/1 -> i_alpha/1  "i_alpha"

== system TestModel_V5_Timing_2024a/Subsystem3/Estimation/Subsystem1 ==
  In Bus Element : Inport  PortName=Ctrl_ScaledISR_In  Element=signal1
  Bus Selector : BusSelector  OutputSignals=signal1,signal2
  Fcn : Fcn  Expr=sin(u(1)*exp(2.3*(-u(2))))
  Iabc_To_Ialphabeta : Subsystem
  Park Transform : mcbcontrolslib/Park Transform  AxisAlignment=D-axis  PhaseInput=Two inputs  ThetaInput=Sine and Cosine electrical position  AngleInput=Per-unit  N_points=1024
      settings: LibrarySourceBlock=mcbhdllib/Controls/Math Transforms/Park Transform
  Pos_Est : Subsystem
  Subsystem : Subsystem
  Terminator : Terminator
  V_AlphaBeta : Subsystem
  di/dt : Subsystem
  emf_AlphaBeta : Subsystem
  Out Bus Element : Outport  PortName=Position_Est  Element=signal1
  Out Bus Element1 : Outport  Port=2  PortName=Speed_Est  Element=signal1
  wires:
  di/dt/1(dia/dt) -> emf_AlphaBeta/3(dia/dt)
  Iabc_To_Ialphabeta/1(i_alpha) -> di/dt/1(i_alpha), [i_alpha]
  emf_AlphaBeta/2(emf_beta) -> Pos_Est/2(emf_beta)
  di/dt/2(dib/dt) -> emf_AlphaBeta/4(dib/dt)
  emf_AlphaBeta/1(emf_alpha) -> Pos_Est/1(emf_alpha)
  V_AlphaBeta/3(V_C) -> Terminator/1
  [i_beta] -> emf_AlphaBeta/2(i_beta)
  [i_alpha] -> emf_AlphaBeta/1(i_alpha)
  V_AlphaBeta/2(V_beta) -> emf_AlphaBeta/6(v_beta)
  ? -> V_AlphaBeta/3(D_b)
  ? -> V_AlphaBeta/1(V_DC)
  V_AlphaBeta/1(V_alpha) -> emf_AlphaBeta/5(v_alpha)
  Iabc_To_Ialphabeta/2(i_beta) -> di/dt/2(i_beta), [i_beta]
  Park Transform/2 -> ?
  Fcn/1 -> ?
  ? -> Iabc_To_Ialphabeta/2(ib)
  Pos_Est/1(Position) -> ?
  ? -> Iabc_To_Ialphabeta/3(ic)
  ? -> Iabc_To_Ialphabeta/1(ia)
  ? -> V_AlphaBeta/4(D_c)
  ? -> V_AlphaBeta/2(D_a)
  Bus Selector/1 -> ?  "<signal1>"
  ? -> Fcn/1
  Park Transform/1 -> ?
  Bus Selector/2 -> ?  "<signal2>"

== system TestModel_V5_Timing_2024a/Open_Loop2/Estimation/Subsystem1/Iabc_To_Ialphabeta ==
  ia : Inport
  ib : Inport  Port=2
  ic : Inport  Port=3
  Add : Sum  Inputs=+--
  Add1 : Sum  Inputs=-+
  Clarke Transform : mcbcontrolslib/Clarke Transform  VariantControl=Variant2  EnPowerInv=off  PhaseInput=Two inputs
      settings: LibrarySourceBlock=mcbhdllib/Controls/Math Transforms/Clarke Transform
  Gain : Gain  Gain=0.5
  Gain1 : Gain  Gain=0.5
  Gain2 : Gain  Gain=2/3
  Gain3 : Gain  Gain=sqrt(3)/2
  Gain4 : Gain  Gain=sqrt(3)/2
  Gain5 : Gain  Gain=2/3
  i_alpha : Outport
  i_beta : Outport  Port=2
  wires:
  Gain3/1 -> Add1/1
  Gain/1 -> Add/2
  ib/1 -> Gain4/1, Gain/1
  Gain5/1 -> i_beta/1  "i_beta"
  ic/1 -> Gain3/1, Gain1/1
  Gain1/1 -> Add/3
  Add1/1 -> Gain5/1
  Add/1 -> Gain2/1
  Gain4/1 -> Add1/2  "i_alpha"
  ia/1 -> Add/1
  Gain2/1 -> i_alpha/1  "i_alpha"

== system TestModel_V5_Timing_2024a/Open_Loop2/Estimation/Subsystem1/Pos_Est ==
  emf_alpha : Inport
  emf_beta : Inport  Port=2
  Gain : Gain
  Trigonometric Function : Trigonometry  Operator=atan2
  Position : Outport
  wires:
  emf_alpha/1 -> Gain/1
  Gain/1 -> Trigonometric Function/1
  emf_beta/1 -> Trigonometric Function/2
  Trigonometric Function/1 -> Position/1

== system TestModel_V5_Timing_2024a/Open_Loop2/Estimation/Subsystem1/Subsystem ==
  1/L : Gain
  Add : Sum  Inputs=+-
  Add1 : Sum
  Add2 : Sum  Inputs=+--
  Add3 : Sum  Inputs=+-
  Ke : Gain
  Ki : Gain
  Rs : Gain
  Unit Delay : UnitDelay  SampleTime=-1  HasFrameUpgradeWarning=on
  wires:
  ? -> Add/1  "i_alpha_meas"
  ? -> Unit Delay/1, Rs/1, Add/2  "i_alpha_est"
  Add/1 -> Ki/1, Ke/1  "i_alpha_tilde"
  Ke/1 -> ?  "d(e_alpha_est)/dt"
  Ki/1 -> Add1/1  "d(e_alpha_est)/dt"
  Add1/1 -> Add3/1  "d(i_alpha_est)/dt"
  ? -> Add2/1  "v_alpha"
  Rs/1 -> Add2/2
  ? -> Add2/3  "e_alpha_est"
  Add2/1 -> 1/L/1
  1/L/1 -> Add1/2
  Unit Delay/1 -> Add3/2

== system TestModel_V5_Timing_2024a/Open_Loop2/Estimation/Subsystem1/V_AlphaBeta ==
  V_DC : Inport
  D_a : Inport  Port=2
  D_b : Inport  Port=3
  D_c : Inport  Port=4
  Add : Sum  Inputs=+-
  Add1 : Sum  Inputs=+-
  Add2 : Sum  Inputs=+-
  Add3 : Sum
  Constant : Constant  Value=0.5
  Constant1 : Constant  Value=0.5
  Constant2 : Constant  Value=0.5
  Gain : Gain  Gain=2
  Gain1 : Gain  Gain=1/sqrt(3)
  Product : Product
  Product1 : Product
  V_alpha : Outport
  V_beta : Outport  Port=2
  V_C : Outport  Port=3
  wires:
  D_a/1 -> Add/1
  Constant/1 -> Add/2
  D_b/1 -> Add1/1
  Constant1/1 -> Add1/2
  D_c/1 -> Add2/1
  Constant2/1 -> Add2/2
  Add/1 -> Product/2
  V_DC/1 -> Product1/1, Product/1
  Product/1 -> Add3/1, V_alpha/1
  Add1/1 -> Product1/2
  Add2/1 -> V_C/1
  Product1/1 -> Gain/1  "V_B"
  Gain/1 -> Add3/2
  Add3/1 -> Gain1/1
  Gain1/1 -> V_beta/1

== system TestModel_V5_Timing_2024a/Open_Loop2/Estimation/Subsystem1/di//dt ==
  i_alpha : Inport
  i_beta : Inport  Port=2
  Subsystem : Subsystem
  Subsystem1 : Subsystem
  dia/dt : Outport
  dib/dt : Outport  Port=2
  wires:
  i_alpha/1 -> Subsystem/1(i_alpha)
  Subsystem/1(dia/dt) -> dia/dt/1
  i_beta/1 -> Subsystem1/1(i_beta)
  Subsystem1/1(dib/dt) -> dib/dt/1

== system TestModel_V5_Timing_2024a/Open_Loop2/Estimation/Subsystem1/emf_AlphaBeta ==
  note: Need to recheck equations:
  i_alpha : Inport
  i_beta : Inport  Port=2
  dia/dt : Inport  Port=3
  dib/dt : Inport  Port=4
  v_alpha : Inport  Port=5
  v_beta : Inport  Port=6
  Add : Sum  Inputs=--+
  Add1 : Sum  Inputs=--+
  Ld : Gain
  Lq : Gain
  Rs : Gain
  Rs1 : Gain
  emf_alpha : Outport
  emf_beta : Outport  Port=2
  wires:
  i_alpha/1 -> Rs/1
  dia/dt/1 -> Ld/1
  Ld/1 -> Add/2
  v_alpha/1 -> Add/3
  Rs/1 -> Add/1
  Add/1 -> emf_alpha/1
  Add1/1 -> emf_beta/1
  Rs1/1 -> Add1/1
  v_beta/1 -> Add1/3
  Lq/1 -> Add1/2
  dib/dt/1 -> Lq/1
  i_beta/1 -> Rs1/1

== system TestModel_V5_Timing_2024a/Subsystem3/Estimation/Subsystem1/Iabc_To_Ialphabeta ==
  ia : Inport
  ib : Inport  Port=2
  ic : Inport  Port=3
  Add : Sum  Inputs=+--
  Add1 : Sum  Inputs=-+
  Clarke Transform : mcbcontrolslib/Clarke Transform  VariantControl=Variant2  EnPowerInv=off  PhaseInput=Two inputs
      settings: LibrarySourceBlock=mcbhdllib/Controls/Math Transforms/Clarke Transform
  Gain : Gain  Gain=0.5
  Gain1 : Gain  Gain=0.5
  Gain2 : Gain  Gain=2/3
  Gain3 : Gain  Gain=sqrt(3)/2
  Gain4 : Gain  Gain=sqrt(3)/2
  Gain5 : Gain  Gain=2/3
  i_alpha : Outport
  i_beta : Outport  Port=2
  wires:
  Gain3/1 -> Add1/1
  Gain/1 -> Add/2
  ib/1 -> Gain4/1, Gain/1
  Gain5/1 -> i_beta/1  "i_beta"
  ic/1 -> Gain3/1, Gain1/1
  Gain1/1 -> Add/3
  Add1/1 -> Gain5/1
  Add/1 -> Gain2/1
  Gain4/1 -> Add1/2  "i_alpha"
  ia/1 -> Add/1
  Gain2/1 -> i_alpha/1  "i_alpha"

== system TestModel_V5_Timing_2024a/Subsystem3/Estimation/Subsystem1/Pos_Est ==
  emf_alpha : Inport
  emf_beta : Inport  Port=2
  Gain : Gain
  Trigonometric Function : Trigonometry  Operator=atan2
  Position : Outport
  wires:
  emf_alpha/1 -> Gain/1
  Gain/1 -> Trigonometric Function/1
  emf_beta/1 -> Trigonometric Function/2
  Trigonometric Function/1 -> Position/1

== system TestModel_V5_Timing_2024a/Subsystem3/Estimation/Subsystem1/Subsystem ==
  1/L : Gain
  Add : Sum  Inputs=+-
  Add1 : Sum
  Add2 : Sum  Inputs=+--
  Add3 : Sum  Inputs=+-
  Ke : Gain
  Ki : Gain
  Rs : Gain
  Unit Delay : UnitDelay  SampleTime=-1  HasFrameUpgradeWarning=on
  wires:
  ? -> Add/1  "i_alpha_meas"
  ? -> Unit Delay/1, Rs/1, Add/2  "i_alpha_est"
  Add/1 -> Ki/1, Ke/1  "i_alpha_tilde"
  Ke/1 -> ?  "d(e_alpha_est)/dt"
  Ki/1 -> Add1/1  "d(e_alpha_est)/dt"
  Add1/1 -> Add3/1  "d(i_alpha_est)/dt"
  ? -> Add2/1  "v_alpha"
  Rs/1 -> Add2/2
  ? -> Add2/3  "e_alpha_est"
  Add2/1 -> 1/L/1
  1/L/1 -> Add1/2
  Unit Delay/1 -> Add3/2

== system TestModel_V5_Timing_2024a/Subsystem3/Estimation/Subsystem1/V_AlphaBeta ==
  V_DC : Inport
  D_a : Inport  Port=2
  D_b : Inport  Port=3
  D_c : Inport  Port=4
  Add : Sum  Inputs=+-
  Add1 : Sum  Inputs=+-
  Add2 : Sum  Inputs=+-
  Add3 : Sum
  Constant : Constant  Value=0.5
  Constant1 : Constant  Value=0.5
  Constant2 : Constant  Value=0.5
  Gain : Gain  Gain=2
  Gain1 : Gain  Gain=1/sqrt(3)
  Product : Product
  Product1 : Product
  V_alpha : Outport
  V_beta : Outport  Port=2
  V_C : Outport  Port=3
  wires:
  D_a/1 -> Add/1
  Constant/1 -> Add/2
  D_b/1 -> Add1/1
  Constant1/1 -> Add1/2
  D_c/1 -> Add2/1
  Constant2/1 -> Add2/2
  Add/1 -> Product/2
  V_DC/1 -> Product1/1, Product/1
  Product/1 -> Add3/1, V_alpha/1
  Add1/1 -> Product1/2
  Add2/1 -> V_C/1
  Product1/1 -> Gain/1  "V_B"
  Gain/1 -> Add3/2
  Add3/1 -> Gain1/1
  Gain1/1 -> V_beta/1

== system TestModel_V5_Timing_2024a/Subsystem3/Estimation/Subsystem1/di//dt ==
  i_alpha : Inport
  i_beta : Inport  Port=2
  Subsystem : Subsystem
  Subsystem1 : Subsystem
  dia/dt : Outport
  dib/dt : Outport  Port=2
  wires:
  i_alpha/1 -> Subsystem/1(i_alpha)
  Subsystem/1(dia/dt) -> dia/dt/1
  i_beta/1 -> Subsystem1/1(i_beta)
  Subsystem1/1(dib/dt) -> dib/dt/1

== system TestModel_V5_Timing_2024a/Subsystem3/Estimation/Subsystem1/emf_AlphaBeta ==
  note: Need to recheck equations:
  i_alpha : Inport
  i_beta : Inport  Port=2
  dia/dt : Inport  Port=3
  dib/dt : Inport  Port=4
  v_alpha : Inport  Port=5
  v_beta : Inport  Port=6
  Add : Sum  Inputs=--+
  Add1 : Sum  Inputs=--+
  Ld : Gain
  Lq : Gain
  Rs : Gain
  Rs1 : Gain
  emf_alpha : Outport
  emf_beta : Outport  Port=2
  wires:
  i_alpha/1 -> Rs/1
  dia/dt/1 -> Ld/1
  Ld/1 -> Add/2
  v_alpha/1 -> Add/3
  Rs/1 -> Add/1
  Add/1 -> emf_alpha/1
  Add1/1 -> emf_beta/1
  Rs1/1 -> Add1/1
  v_beta/1 -> Add1/3
  Lq/1 -> Add1/2
  dib/dt/1 -> Lq/1
  i_beta/1 -> Rs1/1

== system TestModel_V5_Timing_2024a/Open_Loop2/Estimation/Subsystem1/di//dt/Subsystem ==
  i_alpha : Inport
  Add : Sum  Inputs=+-
  Gain : Gain  Gain=1/0.0001
  Unit Delay : UnitDelay  SampleTime=-1  HasFrameUpgradeWarning=on
  dia/dt : Outport
  wires:
  i_alpha/1 -> Unit Delay/1, Add/1
  Unit Delay/1 -> Add/2
  Add/1 -> Gain/1
  Gain/1 -> dia/dt/1

== system TestModel_V5_Timing_2024a/Open_Loop2/Estimation/Subsystem1/di//dt/Subsystem1 ==
  i_beta : Inport
  Add : Sum  Inputs=+-
  Gain : Gain  Gain=1/0.0001
  Unit Delay : UnitDelay  SampleTime=-1  HasFrameUpgradeWarning=on
  dib/dt : Outport
  wires:
  Gain/1 -> dib/dt/1
  Add/1 -> Gain/1
  Unit Delay/1 -> Add/2
  i_beta/1 -> Add/1, Unit Delay/1

== system TestModel_V5_Timing_2024a/Subsystem3/Estimation/Subsystem1/di//dt/Subsystem ==
  i_alpha : Inport
  Add : Sum  Inputs=+-
  Gain : Gain  Gain=1/0.0001
  Unit Delay : UnitDelay  SampleTime=-1  HasFrameUpgradeWarning=on
  dia/dt : Outport
  wires:
  i_alpha/1 -> Unit Delay/1, Add/1
  Unit Delay/1 -> Add/2
  Add/1 -> Gain/1
  Gain/1 -> dia/dt/1

== system TestModel_V5_Timing_2024a/Subsystem3/Estimation/Subsystem1/di//dt/Subsystem1 ==
  i_beta : Inport
  Add : Sum  Inputs=+-
  Gain : Gain  Gain=1/0.0001
  Unit Delay : UnitDelay  SampleTime=-1  HasFrameUpgradeWarning=on
  dib/dt : Outport
  wires:
  Gain/1 -> dib/dt/1
  Add/1 -> Gain/1
  Unit Delay/1 -> Add/2
  i_beta/1 -> Add/1, Unit Delay/1

== matlab function TestModel_V5_Timing_2024a/Subsystem2/Pre_Mag_V1/MATLAB Function2 ==
  data: speed_cmd input; y output; RampUpRate input; RampDownRate input; Ts input
%FileName: Ramp1
%Description: Function to ramp input u1 from output value u2. 
%Inputs: Any Signal Value
%Output: Ramp of input signal until the input value
%Created by: Devi Cheerla
%Created on: 21-08-2024
%Version no: 0.1

% function y = ramp1(u, data)
% u1=u;
% u2=data;
% dy=0.001*4;
% persistent yp;
% if isempty(yp)
%     yp=0;
% elseif (yp==yp && yp~=u2)
%     yp=u2;
% else
% end
% diff = u1-yp;
% 
% if diff>0
%     y=yp+dy;
% elseif diff<0
%     y=yp-dy;
% else
%     y=yp;
% end
% yp=y;
% 
% end


% function y = speed_ramp(speed_cmd,ramp_rate,Ts)
% 
% persistent speed_ref
% 
% % Ts = 1e-6;
% 
% dN = ramp_rate * Ts;
% 
% if isempty(speed_ref)
%     speed_ref = 0;
% end
% 
% err = speed_cmd - speed_ref;
% 
% if abs(err) <= dN
%     speed_ref = speed_cmd;
% elseif err > 0
%     speed_ref = speed_ref + dN;
% else
%     speed_ref = speed_ref - dN;
% end
% 
% y = speed_ref;
% 
% end

function y = speed_ramp(speed_cmd, RampUpRate, RampDownRate, Ts )

persistent speed_ref

% Ts = 1e-3;
% 
% RampUpRate   = 25;
% RampDownRate = 100;

if isempty(speed_ref)
    speed_ref = 0;
end

err = speed_cmd - speed_ref;

if err > 0

    dN = RampUpRate * Ts;

    if err <= dN
        speed_ref = speed_cmd;
    else
        speed_ref = speed_ref + dN;
    end

elseif err < 0

    dN = RampDownRate * Ts;

    if abs(err) <= dN
        speed_ref = speed_cmd;
    else
        speed_ref = speed_ref - dN;
    end

end

y = speed_ref;

end

== matlab function TestModel_V5_Timing_2024a/Subsystem2/Pre_Mag_V1/MATLAB Function4 ==
  data: PreMag_En input; fe input; Vs output; Vs1 input; V_Boost input
function Vs = fcn(PreMag_En, fe,Vs1,V_Boost)
%#codegen

% if fe<6
%     Vs=Vs1+V_Boost;
% else
%     Vs=Vs1;
% end
if PreMag_En == 1
    Vs= V_Boost;
else
    Vs= V_Boost + (400-V_Boost)*fe/50;  %    V_Boost(1+(Vs1/V_Boost)-(fe/50)
end

end

== matlab function TestModel_V5_Timing_2024a/Subsystem2/Pre_Mag_V2/MATLAB Function ==
  data: StartPulse input; PreMag_En output
function PreMag_En = PreMagState(StartPulse)

persistent timer active

Ts = 1e-6;
PreMagTime = 0.2;    % 200 ms

if isempty(timer)
    timer = 0;
    active = 0;
end

if isempty(active)
    timer = 0;
    active = 0;
end

if StartPulse
    %timer = 0;
    active = 1;
    timer = timer + Ts;
    if timer >= PreMagTime
        active = 0;
    end
end

% if active
% 
%     timer = timer + Ts;
% 
%     if timer >= PreMagTime
%         active = 0;
%     end
% 
% end

% if StartPulse
%     timer = 0;
%     active = 1;
% end
% 
% if active
% 
%     timer = timer + Ts;
% 
%     if timer >= PreMagTime
%         active = 0;
%     end
% 
% end

PreMag_En = active;
end

== matlab function TestModel_V5_Timing_2024a/Subsystem2/Pre_Mag_V2/MATLAB Function1 ==
  data: PreMag_En input; Fe_Out output; Fe_Ramp input
function Fe_Out = PreMagState(PreMag_En, Fe_Ramp)

StartupFreq = 3;

if PreMag_En 
    Fe_Out = StartupFreq;
    %Fe_Out = 1.33;
    %Fe_Out = 1;
else
    Fe_Out = max(Fe_Ramp,StartupFreq);
end
end

== matlab function TestModel_V5_Timing_2024a/Subsystem2/Pre_Mag_V2/MATLAB Function2 ==
  data: speed_cmd input; y output; RampUpRate input; RampDownRate input; Ts input
% function y = speed_ramp(StartPulse, speed_cmd, RampUpRate, RampDownRate, Ts)

%%

function y = speed_ramp(speed_cmd, RampUpRate, RampDownRate, Ts )

persistent speed_ref

% Ts = 1e-3;
% 
% RampUpRate   = 25;
% RampDownRate = 100;

if isempty(speed_ref)
    speed_ref = 0;
end

err = speed_cmd - speed_ref;

if err > 0

    dN = RampUpRate * Ts;

    if err <= dN
        speed_ref = speed_cmd;
    else
        speed_ref = speed_ref + dN;
    end

elseif err < 0

    dN = RampDownRate * Ts;

    if abs(err) <= dN
        speed_ref = speed_cmd;
    else
        speed_ref = speed_ref - dN;
    end

end

y = speed_ref;

end

%%
% function y = speed_ramp(StartPulse, speed_cmd, RampUpRate, RampDownRate, Ts)

%persistent speed_ref startup_done

% StartupFreq = 3; % Hz
% 
% if isempty(speed_ref)
%     speed_ref = 0;
%     startup_done = 0;
% end
% 
% % Rising edge of command
% if (StartPulse == 1) && (startup_done == 0)
% 
%     speed_ref = StartupFreq;
%     startup_done = 1;
% 
% end
% 
% % Reset when command removed
% if speed_cmd <= 0
% 
%     speed_ref = 0;
%     startup_done = 0;
% 
% end

% persistent speed_ref
% 
% % Ts = 1e-3;
% % 
% % RampUpRate   = 25;
% % RampDownRate = 100;
% 
% if isempty(speed_ref)
%     speed_ref = 0;
% end
% 
% err = speed_cmd - speed_ref;
% 
% if err > 0
% 
%     speed_ref = min(speed_ref + RampUpRate*Ts, speed_cmd);
% 
% elseif err < 0
% 
%     speed_ref = max(speed_ref - RampDownRate*Ts, speed_cmd);
% 
% end
% 
% y = speed_ref;
% 
% end

%%




%%

%FileName: Ramp1
%Description: Function to ramp input u1 from output value u2. 
%Inputs: Any Signal Value
%Output: Ramp of input signal until the input value
%Created by: Devi Cheerla
%Created on: 21-08-2024
%Version no: 0.1

% function y = ramp1(u, data)
% u1=u;
% u2=data;
% dy=0.001*4;
% persistent yp;
% if isempty(yp)
%     yp=0;
% elseif (yp==yp && yp~=u2)
%     yp=u2;
% else
% end
% diff = u1-yp;
% 
% if diff>0
%     y=yp+dy;
% elseif diff<0
%     y=yp-dy;
% else
%     y=yp;
% end
% yp=y;
% 
% end


% function y = speed_ramp(speed_cmd,ramp_rate,Ts)
% 
% persistent speed_ref
% 
% % Ts = 1e-6;
% 
% dN = ramp_rate * Ts;
% 
% if isempty(speed_ref)
%     speed_ref = 0;
% end
% 
% err = speed_cmd - speed_ref;
% 
% if abs(err) <= dN
%     speed_ref = speed_cmd;
% elseif err > 0
%     speed_ref = speed_ref + dN;
% else
%     speed_ref = speed_ref - dN;
% end
% 
% y = speed_ref;
% 
% end
%%
% function y = speed_ramp(speed_cmd, RampUpRate, RampDownRate, Ts )
% 
% persistent speed_ref
% 
% % Ts = 1e-3;
% % 
% % RampUpRate   = 25;
% % RampDownRate = 100;
% 
% if isempty(speed_ref)
%     speed_ref = 0;
% end
% 
% err = speed_cmd - speed_ref;
% 
% if err > 0
% 
%     dN = RampUpRate * Ts;
% 
%     if err <= dN
%         speed_ref = speed_cmd;
%     else
%         speed_ref = speed_ref + dN;
%     end
% 
% elseif err < 0
% 
%     dN = RampDownRate * Ts;
% 
%     if abs(err) <= dN
%         speed_ref = speed_cmd;
%     else
%         speed_ref = speed_ref - dN;
%     end
% 
% end
% 
% y = speed_ref;
% 
% end
%%

== matlab function TestModel_V5_Timing_2024a/Subsystem2/Pre_Mag_V2/MATLAB Function4 ==
  data: PreMag_En input; fe input; Vs output; Vs1 input; V_Boost input
function Vs = fcn(PreMag_En, fe,Vs1,V_Boost)
%#codegen

% if fe<6
%     Vs=Vs1+V_Boost;
% else
%     Vs=Vs1;
% end
%%
% if PreMag_En == 1
%     Vs= V_Boost;
% else
%     if fe<=0
%         Vs=0;
%     elseif fe<=50
%         Vs=V_Boost + (400-V_Boost)*fe/50;  %    V_Boost(1+(Vs1/V_Boost)-(fe/50);
%     else
%         Vs=400;
%     end
% end
% end
%%

if fe<=0
    Vs = 0;
elseif fe>0 || fe<50
    Vs = V_Boost + (400-V_Boost)*fe/50;  %    V_Boost(1+(Vs1/V_Boost)-(fe/50))
else
    Vs= 400;
end

end
